simulink model "nmm2d"  (R2025a)
settings: Solver=ode15s  StartTime=0.0  StopTime=20  FixedStep=1e-3  MaxStep=ts_max  RelTol=1e-3  AbsTol=1e-4  EnableMultiTasking=on
values from neighbouring files (symbols this model uses):
  c = 0.05    [nmm2d_mInit.m]
  c_jointstop = 0.3 / (pi/180)    (= 17.1887338539)    [nmm2d_mInit.m]
  D12_F = 0.16    [nmm2d_mInit.m]
  D12_S = L_S    (= 0.5)    [nmm2d_mInit.m]
  D12_T = L_T    (= 0.5)    [nmm2d_mInit.m]
  D1G_F = 0.14    [nmm2d_mInit.m]
  D1G_HAT = 0.35    [nmm2d_mInit.m]
  D1G_S = 0.3    [nmm2d_mInit.m]
  D1G_T = 0.3    [nmm2d_mInit.m]
  DeltaThRef = 5e-3    (= 0.005)    [nmm2d_mInit.m]
  eref = 0.04    [nmm2d_mInit.m]
  FmaxVec = [FmaxSOL FmaxTA FmaxGAS FmaxVAS FmaxHAM FmaxGLU FmaxHFL               FmaxSOL FmaxTA FmaxGAS FmaxVAS FmaxHAM FmaxGLU FmaxHFL]'    [nmm2d_mInit.m]
  g = 9.81    [nmm2d_mInit.m]
  GainDeltaTheta = 2 /100*180/pi    (= 1.14591559026)    [nmm2d_cInit.m]
  GainGAS = 1.1/FmaxGAS    [nmm2d_cInit.m]
  GainGLU = 0.5/FmaxGLU    [nmm2d_cInit.m]
  GainHAM = 0.65/FmaxHAM    [nmm2d_cInit.m]
  GainHAMHFL = 4    [nmm2d_cInit.m]
  GainHFL = 0.5    [nmm2d_cInit.m]
  GainKneOverExt = 2    [nmm2d_cInit.m]
  GainSOL = 1.2/FmaxSOL    [nmm2d_cInit.m]
  GainSOLTA = 0.4/FmaxSOL    [nmm2d_cInit.m]
  GainTA = 1.1    [nmm2d_cInit.m]
  GainVAS = 1.2/FmaxVAS    [nmm2d_cInit.m]
  HAT_CG0 = [-D12_F; 0] + Rot120*[L_S;0] + Rot120*Rot230*[-L_T;0]            + Rot120*Rot230*Rot340*[D1G_HAT;0]    [nmm2d_cInit.m]
  In_F = 0.005    [nmm2d_mInit.m]
  In_HAT = 3    [nmm2d_mInit.m]
  In_S = 0.05    [nmm2d_mInit.m]
  In_T = 0.15    [nmm2d_mInit.m]
  K = 5    [nmm2d_mInit.m]
  k_gx = (2*(m_F+m_S+m_T)+m_HAT)*g/0.1    (= 7848)    [nmm2d_mInit.m]
  k_gy = (2*(m_F+m_S+m_T)+m_HAT)*g/0.01    (= 78480)    [nmm2d_mInit.m]
  k_pressure = m_HAT * 9.81 / DeltaThRef    (= 104967)    [nmm2d_mInit.m]
  K_swing = 0.25    [nmm2d_cInit.m]
  KneePh23Offset = 170*pi/180    (= 2.96705972839)    [nmm2d_cInit.m]
  L_F = 0.2    [nmm2d_mInit.m]
  L_HAT = 0.8    [nmm2d_mInit.m]
  L_S = 0.5    [nmm2d_mInit.m]
  L_T = 0.5    [nmm2d_mInit.m]
  LceOffsetHAM = 0.85    [nmm2d_cInit.m]
  LceOffsetHFL = 0.65    [nmm2d_cInit.m]
  LceOffsetTA = 1-0.5*w    [nmm2d_cInit.m]
  LongDelay = 0.020    (= 0.02)    [nmm2d_cInit.m]
  loptGAS = 0.05    [nmm2d_mInit.m]
  loptGLU = 0.11    [nmm2d_mInit.m]
  loptHAM = 0.10    (= 0.1)    [nmm2d_mInit.m]
  loptHFL = 0.11    [nmm2d_mInit.m]
  loptSOL = 0.04    [nmm2d_mInit.m]
  loptTA = 0.06    [nmm2d_mInit.m]
  loptVAS = 0.08    [nmm2d_mInit.m]
  loptVec = [loptSOL loptTA loptGAS loptVAS loptHAM loptGLU loptHFL               loptSOL loptTA loptGAS loptVAS loptHAM loptGLU loptHFL]'    [nmm2d_mInit.m]
  Lphi120 = 85*pi/180    (= 1.4835298642)    [nmm2d_cInit.m]
  Lphi230 = 175*pi/180    (= 3.05432619099)    [nmm2d_cInit.m]
  Lphi340 = 175*pi/180    (= 3.05432619099)    [nmm2d_cInit.m]
  lslackGAS = 0.40    (= 0.4)    [nmm2d_mInit.m]
  lslackGLU = 0.13    [nmm2d_mInit.m]
  lslackHAM = 0.31    [nmm2d_mInit.m]
  lslackHFL = 0.10    (= 0.1)    [nmm2d_mInit.m]
  lslackSOL = 0.26    [nmm2d_mInit.m]
  lslackTA = 0.24    [nmm2d_mInit.m]
  lslackVAS = 0.23    [nmm2d_mInit.m]
  lslackVec = [lslackSOL lslackTA lslackGAS lslackVAS lslackHAM lslackGLU lslackHFL                 lslackSOL lslackTA lslackGAS lslackVAS lslackHAM lslackGLU lslackHFL]'    [nmm2d_mInit.m]
  m_F = 1.25    [nmm2d_mInit.m]
  m_HAT = 53.5    [nmm2d_mInit.m]
  m_S = 3.5    [nmm2d_mInit.m]
  m_T = 8.5    [nmm2d_mInit.m]
  MidDelay = 0.010    (= 0.01)    [nmm2d_cInit.m]
  mu_slide = 0.8    [nmm2d_mInit.m]
  mu_stick = 0.9    [nmm2d_mInit.m]
  N = 1.5    [nmm2d_mInit.m]
  phi12_LowLimit = 70*pi/180    (= 1.2217304764)    [nmm2d_mInit.m]
  phi12_UpLimit = 130*pi/180    (= 2.26892802759)    [nmm2d_mInit.m]
  phi23_UpLimit = 175*pi/180    (= 3.05432619099)    [nmm2d_mInit.m]
  phi34_UpLimit = 230*pi/180    (= 4.01425727959)    [nmm2d_mInit.m]
  phimaxGASa = 110*pi/180    (= 1.91986217719)    [nmm2d_mInit.m]
  phimaxGASk = 140*pi/180    (= 2.44346095279)    [nmm2d_mInit.m]
  phimaxHAMk = 180*pi/180    (= 3.14159265359)    [nmm2d_mInit.m]
  phimaxSOL = 110*pi/180    (= 1.91986217719)    [nmm2d_mInit.m]
  phimaxTA = 80*pi/180    (= 1.3962634016)    [nmm2d_mInit.m]
  phimaxVAS = 165*pi/180    (= 2.87979326579)    [nmm2d_mInit.m]
  phirefGASa = 80*pi/180    (= 1.3962634016)    [nmm2d_mInit.m]
  phirefGASk = 165*pi/180    (= 2.87979326579)    [nmm2d_mInit.m]
  phirefGLU = 150*pi/180    (= 2.61799387799)    [nmm2d_mInit.m]
  phirefHAMh = 155*pi/180    (= 2.70526034059)    [nmm2d_mInit.m]
  phirefHAMk = 180*pi/180    (= 3.14159265359)    [nmm2d_mInit.m]
  phirefHFL = 180*pi/180    (= 3.14159265359)    [nmm2d_mInit.m]
  phirefSOL = 80*pi/180    (= 1.3962634016)    [nmm2d_mInit.m]
  phirefTA = 110*pi/180    (= 1.91986217719)    [nmm2d_mInit.m]
  phirefVAS = 125*pi/180    (= 2.18166156499)    [nmm2d_mInit.m]
  PosGainGG = 1/(30*pi/180)    (= 1.9098593171)    [nmm2d_cInit.m]
  preA = 0.01    [nmm2d_mInit.m]
  PreStimGAS = 0.01    [nmm2d_cInit.m]
  PreStimGG = 0.05    [nmm2d_cInit.m]
  PreStimGLU = 0.01    [nmm2d_cInit.m]
  PreStimHAM = 0.01    [nmm2d_cInit.m]
  PreStimHFL = 0.01    [nmm2d_cInit.m]
  PreStimSOL = 0.01    [nmm2d_cInit.m]
  PreStimTA = 0.01    [nmm2d_cInit.m]
  PreStimVAS = 0.08    [nmm2d_cInit.m]
  rGASa = 0.05    [nmm2d_mInit.m]
  rGASk = 0.05    [nmm2d_mInit.m]
  rGLU = 0.10    (= 0.1)    [nmm2d_mInit.m]
  rHAMh = 0.08    [nmm2d_mInit.m]
  rHAMk = 0.05    [nmm2d_mInit.m]
  rHFL = 0.10    (= 0.1)    [nmm2d_mInit.m]
  rhoGASa = 0.7    [nmm2d_mInit.m]
  rhoGASk = 0.7    [nmm2d_mInit.m]
  rhoGLU = 0.5    [nmm2d_mInit.m]
  rhoHAMh = 0.7    [nmm2d_mInit.m]
  rhoHAMk = 0.7    [nmm2d_mInit.m]
  rhoHFL = 0.5    [nmm2d_mInit.m]
  rhoSOL = 0.5    [nmm2d_mInit.m]
  rhoTA = 0.7    [nmm2d_mInit.m]
  rhoVAS = 0.7    [nmm2d_mInit.m]
  Rphi120 = 90*pi/180    (= 1.57079632679)    [nmm2d_cInit.m]
  Rphi230 = 175*pi/180    (= 3.05432619099)    [nmm2d_cInit.m]
  Rphi340 = 140*pi/180    (= 2.44346095279)    [nmm2d_cInit.m]
  rSOL = 0.05    [nmm2d_mInit.m]
  rTA = 0.04    [nmm2d_mInit.m]
  rVAS = 0.06    [nmm2d_mInit.m]
  ... (+12 more)
undefined symbols (not defined in the file or in its folder): sgn, X, Y, Z
libraries: sm_lib x70, nesl_utility x67, simulink x27, simulink_extras x6
(part 3 of 5)

== system nmm2d/Body Mechanics Layer/Left Thigh Low ==
  Rotate CG to align body w/ x-y plane : sm_lib/Frames and Transforms/Rigid Transform  RotationMethod=StandardAxis  FollAlignAxisA=+X  BaseAlignAxisA=+Y  FollAlignAxisB=+Y  BaseAlignAxisB=+Z  RotationStandardAxis=+X  RotationAngle=-90  RotationAngleUnits=deg  RotationArbitraryAxis=[0 0 1]  RotationSequenceAxes=FollowerAxes  RotationSequence=XYX  RotationSequenceAngles=[0 0 0]  RotationSequenceAnglesUnits=deg  RotationMatrix=[1 0 0; 0 1 0; 0 0 1]  Quaternion=[1 0 0 0]  TranslationMethod=None  TranslationCartesianOffset=[0.25 0 0]  TranslationCartesianOffsetUnits=m  TranslationStandardAxis=+Y  TranslationStandardOffset=-D1G_HAT  TranslationStandardOffsetUnits=m  TranslationROffset=0  TranslationROffsetUnits=m  TranslationThetaOffset=0  TranslationThetaOffsetUnits=deg  TranslationZOffset=0  TranslationZOffsetUnits=m
  Solid : sm_lib/Body Elements/Cylindrical Solid  CylinderRadius=0.03  CylinderRadiusUnits=m  CylinderLength=L_T*ThPos  CylinderLengthUnits=m  ExportEntireGeometry=off  InertiaType=Custom  BasedOnType=Density  Density=2.7  DensityUnits=g/cm^3  Mass=m_T*ThPos  MassUnits=kg  CenterOfMass=[0 0 (D1G_T-L_T/2)*ThPos]  CenterOfMassUnits=m  MomentsOfInertia=In_T*ThPos^3*[1 1 0]  MomentsOfInertiaUnits=kg*m^2  ProductsOfInertia=[0 0 0]  ProductsOfInertiaUnits=kg*m^2  GraphicType=FromGeometry  MarkerShape=Sphere  MarkerSize=10  GraphicVisPropType=SimpleVisualProperties  GraphicDiffuseColor=[1 0.5 0.5]  GraphicOpacity=1.0  GraphicSpecularColor=[0.5 0.5 0.5 1.0]  GraphicAmbientColor=[0.15 0.15 0.15 1.0]  GraphicEmissiveColor=[0 0 0 1.0]  GraphicShininess=75  DoExposeReferenceFrame=off  SerializedFrames=<Frames><Frame><Id>Frame1</Id><Value><Name>CG</Name><Origin><Source>CenterOfMassFrame</Source><FeatureName></FeatureName></Origin><PrimaryAxis><DefinedDirection>+Z</DefinedDirection><Source>ReferenceFrame</Source><SourceDirection>+Z</SourceDirection><FeatureName></FeatureName></PrimaryAxis><SecondaryAxis><DefinedDirection>+X</DefinedDirection><Source>ReferenceFrame</Source><SourceDirection>+X</SourceDirection><FeatureName></FeatureName></SecondaryAxis></Value></Frame></Frames>
  Transform CG to CS2 : sm_lib/Frames and Transforms/Rigid Transform  RotationMethod=None  FollAlignAxisA=+X  BaseAlignAxisA=+Y  FollAlignAxisB=+Y  BaseAlignAxisB=+Z  RotationStandardAxis=+X  RotationAngle=90  RotationAngleUnits=deg  RotationArbitraryAxis=[0 0 1]  RotationSequenceAxes=FollowerAxes  RotationSequence=XYX  RotationSequenceAngles=[0 0 0]  RotationSequenceAnglesUnits=deg  RotationMatrix=[1 0 0; 0 1 0; 0 0 1]  Quaternion=[1 0 0 0]  TranslationMethod=Cartesian  TranslationCartesianOffset=[ 0 D1G_T*ThPos 0]  TranslationCartesianOffsetUnits=m  TranslationStandardAxis=+Y  TranslationStandardOffset=D1G_T*(1-ThPos)  TranslationStandardOffsetUnits=m  TranslationROffset=0  TranslationROffsetUnits=m  TranslationThetaOffset=0  TranslationThetaOffsetUnits=deg  TranslationZOffset=0  TranslationZOffsetUnits=m
  Transform CS1 to CG : sm_lib/Frames and Transforms/Rigid Transform  RotationMethod=None  FollAlignAxisA=+X  BaseAlignAxisA=+Y  FollAlignAxisB=+Y  BaseAlignAxisB=+Z  RotationStandardAxis=+X  RotationAngle=-90  RotationAngleUnits=deg  RotationArbitraryAxis=[0 0 1]  RotationSequenceAxes=FollowerAxes  RotationSequence=XYX  RotationSequenceAngles=[0 0 0]  RotationSequenceAnglesUnits=deg  RotationMatrix=[1 0 0; 0 1 0; 0 0 1]  Quaternion=[1 0 0 0]  TranslationMethod=Cartesian  TranslationCartesianOffset=[0 (D12_T-D1G_T)*ThPos 0]  TranslationCartesianOffsetUnits=m  TranslationStandardAxis=+Y  TranslationStandardOffset=(D12_T-D1G_T)*(1-ThPos)  TranslationStandardOffsetUnits=m  TranslationROffset=0  TranslationROffsetUnits=m  TranslationThetaOffset=0  TranslationThetaOffsetUnits=deg  TranslationZOffset=0  TranslationZOffsetUnits=m
  CS1 : PMIOPort  Side=Left
  CS2 : PMIOPort  Port=2  Side=Right
  connections:
  Solid/LConn1 -- Rotate CG to align body w/ x-y plane/LConn1
  Transform CG to CS2/LConn1 -- Transform CS1 to CG/RConn1 -- Rotate CG to align body w/ x-y plane/RConn1
  Transform CS1 to CG/LConn1 -- CS1/RConn1
  Transform CG to CS2/RConn1 -- CS2/RConn1

== system nmm2d/Body Mechanics Layer/Right Ball Contact ==
  note: Planar Ground Interaction Model
  vBelt : Inport
  " Body Actuator" : nesl_utility/Simulink-PS Converter  PhysicalDomain=network_engine_domain  SubClassName=ps_input  LeftPortType=input  RightPortType=output  PseudoPeriodic=off  Frequencies=[]  NoiseDistribution=none  NoiseParameters=[]  Unit=N  AffineConversion=off  FilteringAndDerivatives=zero  SimscapeFilterOrder=1  InputFilterTimeConstant=.001  UdotUserProvided=0
  " Body Actuator1" : nesl_utility/Simulink-PS Converter  PhysicalDomain=network_engine_domain  SubClassName=ps_input  LeftPortType=input  RightPortType=output  PseudoPeriodic=off  Frequencies=[]  NoiseDistribution=none  NoiseParameters=[]  Unit=N  AffineConversion=off  FilteringAndDerivatives=zero  SimscapeFilterOrder=1  InputFilterTimeConstant=.001  UdotUserProvided=0
  External Force and Torque : sm_lib/Forces and Torques/External Force and Torque  EnableForceX=on  EnableForceY=on  EnableForceZ=off  EnableForce=off  ForceResolutionFrame=World  EnableTorqueX=off  EnableTorqueY=off  EnableTorqueZ=off  EnableTorque=off  TorqueResolutionFrame=AttachedFrame
  Frame Sensor : sm_lib/Frames and Transforms/Transform Sensor  MeasurementFrame=World  RotationSequence=XYX  SenseAngle=off  SenseAxis=off  SenseQ=off  SenseR=off  SenseRotationSequence=off  SenseOmegaX=off  SenseOmegaY=off  SenseOmegaZ=off  SenseOmega=off  SenseQDot=off  SenseRDot=off  SenseRotationSequenceDot=off  SenseAlphaX=off  SenseAlphaY=off  SenseAlphaZ=off  SenseAlpha=off  SenseQDDot=off  SenseRDDot=off  SenseX=on  SenseY=on  SenseZ=off  SenseXYZ=off  SenseRad=off  SenseAzim=off  SenseDist=off  SenseInc=off  SenseXDot=on  SenseYDot=on  SenseZDot=off  SenseXYZDot=off  SenseRadDot=off  SenseAzimDot=off  SenseDistDot=off  SenseIncDot=off  SenseXDDot=off  SenseYDDot=off  SenseZDDot=off  SenseXYZDDot=off  SenseRadDDot=off  SenseAzimDDot=off  SenseDistDDot=off  SenseIncDDot=off
  Ground Friction Model : Subsystem
  Mux : Mux  Inputs=2
  PS-Simulink Converter : nesl_utility/PS-Simulink Converter  PhysicalDomain=network_engine_domain  SubClassName=ps_output  LeftPortType=input  RightPortType=output  PseudoPeriodic=off  Frequencies=[]  VectorFormat=1-D array  Unit=m  AffineConversion=off
  PS-Simulink Converter1 : nesl_utility/PS-Simulink Converter  PhysicalDomain=network_engine_domain  SubClassName=ps_output  LeftPortType=input  RightPortType=output  PseudoPeriodic=off  Frequencies=[]  VectorFormat=1-D array  Unit=m  AffineConversion=off
  PS-Simulink Converter2 : nesl_utility/PS-Simulink Converter  PhysicalDomain=network_engine_domain  SubClassName=ps_output  LeftPortType=input  RightPortType=output  PseudoPeriodic=off  Frequencies=[]  VectorFormat=1-D array  Unit=m/s  AffineConversion=off
  PS-Simulink Converter3 : nesl_utility/PS-Simulink Converter  PhysicalDomain=network_engine_domain  SubClassName=ps_output  LeftPortType=input  RightPortType=output  PseudoPeriodic=off  Frequencies=[]  VectorFormat=1-D array  Unit=m/s  AffineConversion=off
  Sum : Sum  Inputs=-+|
  Terminator : Terminator
  World Frame : sm_lib/Frames and Transforms/World Frame
  skin contact sensor : simulink/Logic and Bit Operations/Compare To Zero  relop=<=  OutDataTypeStr=boolean
  yGround : Constant  Value=0
  F : PMIOPort  Side=Left
  LHeelCnt : Outport
  GRF [N N] : Outport  Port=2
  wires:
  PS-Simulink Converter2/1 -> Ground Friction Model/4(vx [m/s])
  PS-Simulink Converter/1 -> Ground Friction Model/3(x [m])
  PS-Simulink Converter3/1 -> Ground Friction Model/2(vy [m/s])
  PS-Simulink Converter1/1 -> Sum/2
  Sum/1 -> skin contact sensor/1, Ground Friction Model/1(dy [m])
  yGround/1 -> Sum/1
  Mux/1 -> GRF [N N]/1
  skin contact sensor/1 -> LHeelCnt/1, Ground Friction Model/Enable
  Ground Friction Model/1(Fy_Ground[N]) -> Mux/2, " Body Actuator1"/1
  Ground Friction Model/2(Fx_Friction [N]) -> Mux/1, " Body Actuator"/1
  Ground Friction Model/3(Stiction!) -> Terminator/1
  vBelt/1 -> Ground Friction Model/5(vBelt [m/s])
  connections:
  World Frame/RConn1 -- Frame Sensor/LConn1
  PS-Simulink Converter2/LConn1 -- Frame Sensor/RConn4
  PS-Simulink Converter1/LConn1 -- Frame Sensor/RConn3
  Frame Sensor/RConn2 -- PS-Simulink Converter/LConn1
  PS-Simulink Converter3/LConn1 -- Frame Sensor/RConn5
  External Force and Torque/RConn1 -- Frame Sensor/RConn1 -- F/RConn1
  External Force and Torque/LConn2 -- " Body Actuator1"/RConn1
  External Force and Torque/LConn1 -- " Body Actuator"/RConn1

== system nmm2d/Body Mechanics Layer/Right Heel Contact ==
  note: Planar Ground Interaction Model
  vBelt : Inport
  " Body Actuator" : nesl_utility/Simulink-PS Converter  PhysicalDomain=network_engine_domain  SubClassName=ps_input  LeftPortType=input  RightPortType=output  PseudoPeriodic=off  Frequencies=[]  NoiseDistribution=none  NoiseParameters=[]  Unit=N  AffineConversion=off  FilteringAndDerivatives=zero  SimscapeFilterOrder=1  InputFilterTimeConstant=.001  UdotUserProvided=0
  " Body Actuator1" : nesl_utility/Simulink-PS Converter  PhysicalDomain=network_engine_domain  SubClassName=ps_input  LeftPortType=input  RightPortType=output  PseudoPeriodic=off  Frequencies=[]  NoiseDistribution=none  NoiseParameters=[]  Unit=N  AffineConversion=off  FilteringAndDerivatives=zero  SimscapeFilterOrder=1  InputFilterTimeConstant=.001  UdotUserProvided=0
  External Force and Torque : sm_lib/Forces and Torques/External Force and Torque  EnableForceX=on  EnableForceY=on  EnableForceZ=off  EnableForce=off  ForceResolutionFrame=World  EnableTorqueX=off  EnableTorqueY=off  EnableTorqueZ=off  EnableTorque=off  TorqueResolutionFrame=AttachedFrame
  Frame Sensor : sm_lib/Frames and Transforms/Transform Sensor  MeasurementFrame=World  RotationSequence=XYX  SenseAngle=off  SenseAxis=off  SenseQ=off  SenseR=off  SenseRotationSequence=off  SenseOmegaX=off  SenseOmegaY=off  SenseOmegaZ=off  SenseOmega=off  SenseQDot=off  SenseRDot=off  SenseRotationSequenceDot=off  SenseAlphaX=off  SenseAlphaY=off  SenseAlphaZ=off  SenseAlpha=off  SenseQDDot=off  SenseRDDot=off  SenseX=on  SenseY=on  SenseZ=off  SenseXYZ=off  SenseRad=off  SenseAzim=off  SenseDist=off  SenseInc=off  SenseXDot=on  SenseYDot=on  SenseZDot=off  SenseXYZDot=off  SenseRadDot=off  SenseAzimDot=off  SenseDistDot=off  SenseIncDot=off  SenseXDDot=off  SenseYDDot=off  SenseZDDot=off  SenseXYZDDot=off  SenseRadDDot=off  SenseAzimDDot=off  SenseDistDDot=off  SenseIncDDot=off
  Ground Friction Model : Subsystem
  Mux : Mux  Inputs=2
  PS-Simulink Converter : nesl_utility/PS-Simulink Converter  PhysicalDomain=network_engine_domain  SubClassName=ps_output  LeftPortType=input  RightPortType=output  PseudoPeriodic=off  Frequencies=[]  VectorFormat=1-D array  Unit=m  AffineConversion=off
  PS-Simulink Converter1 : nesl_utility/PS-Simulink Converter  PhysicalDomain=network_engine_domain  SubClassName=ps_output  LeftPortType=input  RightPortType=output  PseudoPeriodic=off  Frequencies=[]  VectorFormat=1-D array  Unit=m  AffineConversion=off
  PS-Simulink Converter2 : nesl_utility/PS-Simulink Converter  PhysicalDomain=network_engine_domain  SubClassName=ps_output  LeftPortType=input  RightPortType=output  PseudoPeriodic=off  Frequencies=[]  VectorFormat=1-D array  Unit=m/s  AffineConversion=off
  PS-Simulink Converter3 : nesl_utility/PS-Simulink Converter  PhysicalDomain=network_engine_domain  SubClassName=ps_output  LeftPortType=input  RightPortType=output  PseudoPeriodic=off  Frequencies=[]  VectorFormat=1-D array  Unit=m/s  AffineConversion=off
  Sum : Sum  Inputs=-+|
  Terminator : Terminator
  World Frame : sm_lib/Frames and Transforms/World Frame
  skin contact sensor : simulink/Logic and Bit Operations/Compare To Zero  relop=<=  OutDataTypeStr=boolean
  yGround : Constant  Value=0
  F : PMIOPort  Side=Left
  LHeelCnt : Outport
  GRF [N N] : Outport  Port=2
  wires:
  vBelt/1 -> Ground Friction Model/5(vBelt [m/s])
  Ground Friction Model/3(Stiction!) -> Terminator/1
  Ground Friction Model/2(Fx_Friction [N]) -> " Body Actuator"/1, Mux/1
  Ground Friction Model/1(Fy_Ground[N]) -> " Body Actuator1"/1, Mux/2
  skin contact sensor/1 -> Ground Friction Model/Enable, LHeelCnt/1
  Mux/1 -> GRF [N N]/1
  yGround/1 -> Sum/1
  Sum/1 -> Ground Friction Model/1(dy [m]), skin contact sensor/1
  PS-Simulink Converter1/1 -> Sum/2
  PS-Simulink Converter3/1 -> Ground Friction Model/2(vy [m/s])
  PS-Simulink Converter/1 -> Ground Friction Model/3(x [m])
  PS-Simulink Converter2/1 -> Ground Friction Model/4(vx [m/s])
  connections:
  External Force and Torque/LConn1 -- " Body Actuator"/RConn1
  External Force and Torque/LConn2 -- " Body Actuator1"/RConn1
  F/RConn1 -- Frame Sensor/RConn1 -- External Force and Torque/RConn1
  PS-Simulink Converter3/LConn1 -- Frame Sensor/RConn5
  Frame Sensor/RConn2 -- PS-Simulink Converter/LConn1
  PS-Simulink Converter1/LConn1 -- Frame Sensor/RConn3
  PS-Simulink Converter2/LConn1 -- Frame Sensor/RConn4
  World Frame/RConn1 -- Frame Sensor/LConn1

== system nmm2d/Body Mechanics Layer/Right Foot ==
  Rotate CG to align body w/ x-y plane : sm_lib/Frames and Transforms/Rigid Transform  RotationMethod=StandardAxis  FollAlignAxisA=+X  BaseAlignAxisA=+Y  FollAlignAxisB=+Y  BaseAlignAxisB=+Z  RotationStandardAxis=+X  RotationAngle=-90  RotationAngleUnits=deg  RotationArbitraryAxis=[0 0 1]  RotationSequenceAxes=FollowerAxes  RotationSequence=XYX  RotationSequenceAngles=[0 0 0]  RotationSequenceAnglesUnits=deg  RotationMatrix=[1 0 0; 0 1 0; 0 0 1]  Quaternion=[1 0 0 0]  TranslationMethod=None  TranslationCartesianOffset=[0.25 0 0]  TranslationCartesianOffsetUnits=m  TranslationStandardAxis=+Y  TranslationStandardOffset=-D1G_HAT  TranslationStandardOffsetUnits=m  TranslationROffset=0  TranslationROffsetUnits=m  TranslationThetaOffset=0  TranslationThetaOffsetUnits=deg  TranslationZOffset=0  TranslationZOffsetUnits=m
  Solid : sm_lib/Body Elements/Cylindrical Solid  CylinderRadius=0.01  CylinderRadiusUnits=m  CylinderLength=L_F  CylinderLengthUnits=m  ExportEntireGeometry=off  InertiaType=Custom  BasedOnType=Density  Density=2.7  DensityUnits=g/cm^3  Mass=m_F  MassUnits=kg  CenterOfMass=[0 0 D1G_F-L_F/2]  CenterOfMassUnits=m  MomentsOfInertia=In_F*[1 1 0]  MomentsOfInertiaUnits=kg*m^2  ProductsOfInertia=[0 0 0]  ProductsOfInertiaUnits=kg*m^2  GraphicType=FromGeometry  MarkerShape=Sphere  MarkerSize=10  GraphicVisPropType=SimpleVisualProperties  GraphicDiffuseColor=[1 0.5 0.5]  GraphicOpacity=1.0  GraphicSpecularColor=[0.5 0.5 0.5 1.0]  GraphicAmbientColor=[0.15 0.15 0.15 1.0]  GraphicEmissiveColor=[0 0 0 1.0]  GraphicShininess=75  DoExposeReferenceFrame=off  SerializedFrames=<Frames><Frame><Id>Frame1</Id><Value><Name>CG</Name><Origin><Source>CenterOfMassFrame</Source><FeatureName></FeatureName></Origin><PrimaryAxis><DefinedDirection>+Z</DefinedDirection><Source>ReferenceFrame</Source><SourceDirection>+Z</SourceDirection><FeatureName></FeatureName></PrimaryAxis><SecondaryAxis><DefinedDirection>+X</DefinedDirection><Source>ReferenceFrame</Source><SourceDirection>+X</SourceDirection><FeatureName></FeatureName></SecondaryAxis></Value></Frame></Frames>
  Transform CG to CS2 : sm_lib/Frames and Transforms/Rigid Transform  RotationMethod=None  FollAlignAxisA=+X  BaseAlignAxisA=+Y  FollAlignAxisB=+Y  BaseAlignAxisB=+Z  RotationStandardAxis=+X  RotationAngle=90  RotationAngleUnits=deg  RotationArbitraryAxis=[0 0 1]  RotationSequenceAxes=FollowerAxes  RotationSequence=XYX  RotationSequenceAngles=[0 0 0]  RotationSequenceAnglesUnits=deg  RotationMatrix=[1 0 0; 0 1 0; 0 0 1]  Quaternion=[1 0 0 0]  TranslationMethod=Cartesian  TranslationCartesianOffset=[ 0 D1G_F 0]  TranslationCartesianOffsetUnits=m  TranslationStandardAxis=+Y  TranslationStandardOffset=D1G_T*(1-ThPos)  TranslationStandardOffsetUnits=m  TranslationROffset=0  TranslationROffsetUnits=m  TranslationThetaOffset=0  TranslationThetaOffsetUnits=deg  TranslationZOffset=0  TranslationZOffsetUnits=m
  Transform CS1 to CG : sm_lib/Frames and Transforms/Rigid Transform  RotationMethod=None  FollAlignAxisA=+X  BaseAlignAxisA=+Y  FollAlignAxisB=+Y  BaseAlignAxisB=+Z  RotationStandardAxis=+X  RotationAngle=-90  RotationAngleUnits=deg  RotationArbitraryAxis=[0 0 1]  RotationSequenceAxes=FollowerAxes  RotationSequence=XYX  RotationSequenceAngles=[0 0 0]  RotationSequenceAnglesUnits=deg  RotationMatrix=[1 0 0; 0 1 0; 0 0 1]  Quaternion=[1 0 0 0]  TranslationMethod=Cartesian  TranslationCartesianOffset=[0 (D12_F-D1G_F) 0]  TranslationCartesianOffsetUnits=m  TranslationStandardAxis=+Y  TranslationStandardOffset=(D12_T-D1G_T)*(1-ThPos)  TranslationStandardOffsetUnits=m  TranslationROffset=0  TranslationROffsetUnits=m  TranslationThetaOffset=0  TranslationThetaOffsetUnits=deg  TranslationZOffset=0  TranslationZOffsetUnits=m
  Transform CS1 to CS3 : sm_lib/Frames and Transforms/Rigid Transform  RotationMethod=None  FollAlignAxisA=+X  BaseAlignAxisA=+Y  FollAlignAxisB=+Y  BaseAlignAxisB=+Z  RotationStandardAxis=+X  RotationAngle=-90  RotationAngleUnits=deg  RotationArbitraryAxis=[0 0 1]  RotationSequenceAxes=FollowerAxes  RotationSequence=XYX  RotationSequenceAngles=[0 0 0]  RotationSequenceAnglesUnits=deg  RotationMatrix=[1 0 0; 0 1 0; 0 0 1]  Quaternion=[1 0 0 0]  TranslationMethod=Cartesian  TranslationCartesianOffset=[0 -(L_F-D12_F) 0]  TranslationCartesianOffsetUnits=m  TranslationStandardAxis=+Y  TranslationStandardOffset=(D12_T-D1G_T)*(1-ThPos)  TranslationStandardOffsetUnits=m  TranslationROffset=0  TranslationROffsetUnits=m  TranslationThetaOffset=0  TranslationThetaOffsetUnits=deg  TranslationZOffset=0  TranslationZOffsetUnits=m
  CS1 : PMIOPort  Side=Left
  CS2 : PMIOPort  Port=2  Side=Right
  CS3 : PMIOPort  Port=3  Side=Left
  connections:
  Transform CS1 to CS3/RConn1 -- CS3/RConn1
  Solid/LConn1 -- Rotate CG to align body w/ x-y plane/LConn1
  Rotate CG to align body w/ x-y plane/RConn1 -- Transform CG to CS2/LConn1 -- Transform CS1 to CG/RConn1
  CS1/RConn1 -- Transform CS1 to CS3/LConn1 -- Transform CS1 to CG/LConn1
  Transform CG to CS2/RConn1 -- CS2/RConn1

== system nmm2d/Body Mechanics Layer/Right Force Plate ==
  "GRF_Ball [N N] " : Inport
  GRF_Heel [N N] : Inport  Port=2
  Enable : EnablePort  StatesWhenEnabling=reset
  Fcn : Fcn  Expr=u(1)/(u(2)+eps)
  Mux : Mux  Inputs=3
  Mux1 : Mux  Inputs=2
  Selector : Selector  InputPortWidth=2  IndexOptions=Index vector (dialog)  Indices=2  OutputSizes=1
  Selector1 : Selector  InputPortWidth=2  IndexOptions=Index vector (dialog)  Indices=2  OutputSizes=1
  Sum1 : Sum
  GRFs : Outport  OutputWhenDisabled=reset  InitialOutput=0
  COP : Outport  Port=2  OutputWhenDisabled=reset  InitialOutput=0
  wires:
  Fcn/1 -> COP/1
  Mux1/1 -> Fcn/1
  Mux/1 -> GRFs/1
  Sum1/1 -> Selector/1, Mux/2
  GRF_Heel [N N]/1 -> Mux/3, Sum1/2
  "GRF_Ball [N N] "/1 -> Selector1/1, Mux/1, Sum1/1
  Selector1/1 -> Mux1/1
  Selector/1 -> Mux1/2

== system nmm2d/Body Mechanics Layer/Right Shank ==
  Rotate CG to align body w/ x-y plane : sm_lib/Frames and Transforms/Rigid Transform  RotationMethod=StandardAxis  FollAlignAxisA=+X  BaseAlignAxisA=+Y  FollAlignAxisB=+Y  BaseAlignAxisB=+Z  RotationStandardAxis=+X  RotationAngle=-90  RotationAngleUnits=deg  RotationArbitraryAxis=[0 0 1]  RotationSequenceAxes=FollowerAxes  RotationSequence=XYX  RotationSequenceAngles=[0 0 0]  RotationSequenceAnglesUnits=deg  RotationMatrix=[1 0 0; 0 1 0; 0 0 1]  Quaternion=[1 0 0 0]  TranslationMethod=None  TranslationCartesianOffset=[0.25 0 0]  TranslationCartesianOffsetUnits=m  TranslationStandardAxis=+Y  TranslationStandardOffset=-D1G_HAT  TranslationStandardOffsetUnits=m  TranslationROffset=0  TranslationROffsetUnits=m  TranslationThetaOffset=0  TranslationThetaOffsetUnits=deg  TranslationZOffset=0  TranslationZOffsetUnits=m
  Solid : sm_lib/Body Elements/Cylindrical Solid  CylinderRadius=0.02  CylinderRadiusUnits=m  CylinderLength=L_S  CylinderLengthUnits=m  ExportEntireGeometry=off  InertiaType=Custom  BasedOnType=Density  Density=2.7  DensityUnits=g/cm^3  Mass=m_S  MassUnits=kg  CenterOfMass=[0 0 L_S/2-D1G_S]  CenterOfMassUnits=m  MomentsOfInertia=In_S*[1 1 0]  MomentsOfInertiaUnits=kg*m^2  ProductsOfInertia=[0 0 0]  ProductsOfInertiaUnits=kg*m^2  GraphicType=FromGeometry  MarkerShape=Sphere  MarkerSize=10  GraphicVisPropType=SimpleVisualProperties  GraphicDiffuseColor=[1 0.5 0.5]  GraphicOpacity=1.0  GraphicSpecularColor=[0.5 0.5 0.5 1.0]  GraphicAmbientColor=[0.15 0.15 0.15 1.0]  GraphicEmissiveColor=[0 0 0 1.0]  GraphicShininess=75  DoExposeReferenceFrame=off  SerializedFrames=<Frames><Frame><Id>Frame1</Id><Value><Name>CG</Name><Origin><Source>CenterOfMassFrame</Source><FeatureName></FeatureName></Origin><PrimaryAxis><DefinedDirection>+Z</DefinedDirection><Source>ReferenceFrame</Source><SourceDirection>+Z</SourceDirection><FeatureName></FeatureName></PrimaryAxis><SecondaryAxis><DefinedDirection>+X</DefinedDirection><Source>ReferenceFrame</Source><SourceDirection>+X</SourceDirection><FeatureName></FeatureName></SecondaryAxis></Value></Frame></Frames>
  Transform CG to CS2 : sm_lib/Frames and Transforms/Rigid Transform  RotationMethod=None  FollAlignAxisA=+X  BaseAlignAxisA=+Y  FollAlignAxisB=+Y  BaseAlignAxisB=+Z  RotationStandardAxis=+X  RotationAngle=90  RotationAngleUnits=deg  RotationArbitraryAxis=[0 0 1]  RotationSequenceAxes=FollowerAxes  RotationSequence=XYX  RotationSequenceAngles=[0 0 0]  RotationSequenceAnglesUnits=deg  RotationMatrix=[1 0 0; 0 1 0; 0 0 1]  Quaternion=[1 0 0 0]  TranslationMethod=Cartesian  TranslationCartesianOffset=[ 0 -D1G_S 0]  TranslationCartesianOffsetUnits=m  TranslationStandardAxis=+Y  TranslationStandardOffset=D1G_T*(1-ThPos)  TranslationStandardOffsetUnits=m  TranslationROffset=0  TranslationROffsetUnits=m  TranslationThetaOffset=0  TranslationThetaOffsetUnits=deg  TranslationZOffset=0  TranslationZOffsetUnits=m
  Transform CS1 to CG : sm_lib/Frames and Transforms/Rigid Transform  RotationMethod=None  FollAlignAxisA=+X  BaseAlignAxisA=+Y  FollAlignAxisB=+Y  BaseAlignAxisB=+Z  RotationStandardAxis=+X  RotationAngle=-90  RotationAngleUnits=deg  RotationArbitraryAxis=[0 0 1]  RotationSequenceAxes=FollowerAxes  RotationSequence=XYX  RotationSequenceAngles=[0 0 0]  RotationSequenceAnglesUnits=deg  RotationMatrix=[1 0 0; 0 1 0; 0 0 1]  Quaternion=[1 0 0 0]  TranslationMethod=Cartesian  TranslationCartesianOffset=[0 -(D12_S-D1G_S) 0]  TranslationCartesianOffsetUnits=m  TranslationStandardAxis=+Y  TranslationStandardOffset=(D12_T-D1G_T)*(1-ThPos)  TranslationStandardOffsetUnits=m  TranslationROffset=0  TranslationROffsetUnits=m  TranslationThetaOffset=0  TranslationThetaOffsetUnits=deg  TranslationZOffset=0  TranslationZOffsetUnits=m
  CS1 : PMIOPort  Side=Left
  CS2 : PMIOPort  Port=2  Side=Right
  connections:
  Transform CG to CS2/RConn1 -- CS2/RConn1
  Transform CS1 to CG/LConn1 -- CS1/RConn1
  Rotate CG to align body w/ x-y plane/RConn1 -- Transform CS1 to CG/RConn1 -- Transform CG to CS2/LConn1
  Solid/LConn1 -- Rotate CG to align body w/ x-y plane/LConn1

== system nmm2d/Body Mechanics Layer/Right Thigh Sensor Sheet ==
  note: Inner Segment Pressure Sheet
  Gain3 : Gain  Gain=k_pressure
  Gain4 : Gain  Gain=1/v_max_pressure
  Inner Thigh Shift Joint : sm_lib/Joints/Prismatic Joint  JointMode=Normal  CompositeWrenchDir=FollowerOnBase  CompositeWrenchFrame=BaseFrame  SenseConstraintForce=off  SenseConstraintTorque=off  SenseTotalForce=off  SenseTotalTorque=off  PositionTargetSpecify=on  PositionTargetPriority=High  PositionTargetValue=0  PositionTargetValueUnits=m  VelocityTargetSpecify=on  VelocityTargetPriority=High  VelocityTargetValue=0  VelocityTargetValueUnits=m/s  EquilibriumPosition=0  EquilibriumPositionUnits=m  SpringStiffness=0  SpringStiffnessUnits=N/m  DampingCoefficient=0  DampingCoefficientUnits=N/(m/s)  LowerLimitSpecify=off  LowerLimitBound=-1  LowerLimitBoundUnits=m  LowerLimitStiffness=1e6  LowerLimitStiffnessUnits=N/m  LowerLimitDamping=1e3  LowerLimitDampingUnits=N/(m/s)  LowerLimitTransitionRegionWidth=1e-4  LowerLimitTransitionRegionWidthUnits=m  UpperLimitSpecify=off  UpperLimitBound=1  UpperLimitBoundUnits=m  UpperLimitStiffness=1e6  UpperLimitStiffnessUnits=N/m  UpperLimitDamping=1e3  UpperLimitDampingUnits=N/(m/s)  UpperLimitTransitionRegionWidth=1e-4  UpperLimitTransitionRegionWidthUnits=m  TorqueActuationMode=InputTorque  MotionActuationMode=ComputedMotion  SensePosition=on  SenseVelocity=on  SenseAcceleration=off  SenseTorqueForce=off  SenseLowerLimitTorqueForce=off  SenseUpperLimitTorqueForce=off
  Mux1 : Mux  Inputs=2
  Pressure Sheet Reaction Force : Fcn  Expr=-u(1) * (1+sgn(u(1))*u(2))
  Rotate back to y-axis : sm_lib/Frames and Transforms/Rigid Transform  RotationMethod=StandardAxis  FollAlignAxisA=+X  BaseAlignAxisA=+Y  FollAlignAxisB=+Y  BaseAlignAxisB=+Z  RotationStandardAxis=+X  RotationAngle=-90  RotationAngleUnits=deg  RotationArbitraryAxis=[0 0 1]  RotationSequenceAxes=FollowerAxes  RotationSequence=XYX  RotationSequenceAngles=[0 0 0]  RotationSequenceAnglesUnits=deg  RotationMatrix=[1 0 0; 0 1 0; 0 0 1]  Quaternion=[1 0 0 0]  TranslationMethod=None  TranslationCartesianOffset=[0 0 0]  TranslationCartesianOffsetUnits=m  TranslationStandardAxis=+Z  TranslationStandardOffset=0  TranslationStandardOffsetUnits=m  TranslationROffset=0  TranslationROffsetUnits=m  TranslationThetaOffset=0  TranslationThetaOffsetUnits=deg  TranslationZOffset=0  TranslationZOffsetUnits=m
  Rotate into z-axis : sm_lib/Frames and Transforms/Rigid Transform  RotationMethod=StandardAxis  FollAlignAxisA=+X  BaseAlignAxisA=+Y  FollAlignAxisB=+Y  BaseAlignAxisB=+Z  RotationStandardAxis=+X  RotationAngle=90  RotationAngleUnits=deg  RotationArbitraryAxis=[0 0 1]  RotationSequenceAxes=FollowerAxes  RotationSequence=XYX  RotationSequenceAngles=[0 0 0]  RotationSequenceAnglesUnits=deg  RotationMatrix=[1 0 0; 0 1 0; 0 0 1]  Quaternion=[1 0 0 0]  TranslationMethod=None  TranslationCartesianOffset=[0 0 0]  TranslationCartesianOffsetUnits=m  TranslationStandardAxis=+Z  TranslationStandardOffset=0  TranslationStandardOffsetUnits=m  TranslationROffset=0  TranslationROffsetUnits=m  TranslationThetaOffset=0  TranslationThetaOffsetUnits=deg  TranslationZOffset=0  TranslationZOffsetUnits=m
  Thigh Actuator : nesl_utility/Simulink-PS Converter  PhysicalDomain=network_engine_domain  SubClassName=ps_input  LeftPortType=input  RightPortType=output  PseudoPeriodic=off  Frequencies=[]  NoiseDistribution=none  NoiseParameters=[]  Unit=N  AffineConversion=off  FilteringAndDerivatives=zero  SimscapeFilterOrder=1  InputFilterTimeConstant=.001  UdotUserProvided=0
  Thigh Pos Sensor : nesl_utility/PS-Simulink Converter  PhysicalDomain=network_engine_domain  SubClassName=ps_output  LeftPortType=input  RightPortType=output  PseudoPeriodic=off  Frequencies=[]  VectorFormat=1-D array  Unit=m  AffineConversion=off
  Thigh Vel Sensor : nesl_utility/PS-Simulink Converter  PhysicalDomain=network_engine_domain  SubClassName=ps_output  LeftPortType=input  RightPortType=output  PseudoPeriodic=off  Frequencies=[]  VectorFormat=1-D array  Unit=m/s  AffineConversion=off
  F : PMIOPort  Side=Right
  B : PMIOPort  Port=2  Side=Left
  dx : Outport
  wires:
  Gain3/1 -> Mux1/1
  Gain4/1 -> Mux1/2
  Mux1/1 -> Pressure Sheet Reaction Force/1
  Thigh Vel Sensor/1 -> Gain4/1
  Pressure Sheet Reaction Force/1 -> Thigh Actuator/1
  Thigh Pos Sensor/1 -> Gain3/1, dx/1
  connections:
  F/RConn1 -- Rotate back to y-axis/RConn1
  B/RConn1 -- Rotate into z-axis/LConn1
  Inner Thigh Shift Joint/RConn2 -- Thigh Pos Sensor/LConn1
  Thigh Vel Sensor/LConn1 -- Inner Thigh Shift Joint/RConn3
  Thigh Actuator/RConn1 -- Inner Thigh Shift Joint/LConn2
  Rotate into z-axis/RConn1 -- Inner Thigh Shift Joint/LConn1
  Rotate back to y-axis/LConn1 -- Inner Thigh Shift Joint/RConn1

== system nmm2d/Body Mechanics Layer/Right Thigh High ==
  Rotate CG to align body w/ x-y plane : sm_lib/Frames and Transforms/Rigid Transform  RotationMethod=StandardAxis  FollAlignAxisA=+X  BaseAlignAxisA=+Y  FollAlignAxisB=+Y  BaseAlignAxisB=+Z  RotationStandardAxis=+X  RotationAngle=-90  RotationAngleUnits=deg  RotationArbitraryAxis=[0 0 1]  RotationSequenceAxes=FollowerAxes  RotationSequence=XYX  RotationSequenceAngles=[0 0 0]  RotationSequenceAnglesUnits=deg  RotationMatrix=[1 0 0; 0 1 0; 0 0 1]  Quaternion=[1 0 0 0]  TranslationMethod=None  TranslationCartesianOffset=[0.25 0 0]  TranslationCartesianOffsetUnits=m  TranslationStandardAxis=+Y  TranslationStandardOffset=-D1G_HAT  TranslationStandardOffsetUnits=m  TranslationROffset=0  TranslationROffsetUnits=m  TranslationThetaOffset=0  TranslationThetaOffsetUnits=deg  TranslationZOffset=0  TranslationZOffsetUnits=m
  Solid : sm_lib/Body Elements/Cylindrical Solid  CylinderRadius=0.03  CylinderRadiusUnits=m  CylinderLength=L_T*(1-ThPos)  CylinderLengthUnits=m  ExportEntireGeometry=off  InertiaType=Custom  BasedOnType=Density  Density=2.7  DensityUnits=g/cm^3  Mass=m_T*(1-ThPos)  MassUnits=kg  CenterOfMass=[0 0 (D1G_T-L_T/2)*(1-ThPos)]  CenterOfMassUnits=m  MomentsOfInertia=In_T*(1-ThPos)^3*[1 1 0]  MomentsOfInertiaUnits=kg*m^2  ProductsOfInertia=[0 0 0]  ProductsOfInertiaUnits=kg*m^2  GraphicType=FromGeometry  MarkerShape=Sphere  MarkerSize=10  GraphicVisPropType=SimpleVisualProperties  GraphicDiffuseColor=[1 0.5 0.5]  GraphicOpacity=1.0  GraphicSpecularColor=[0.5 0.5 0.5 1.0]  GraphicAmbientColor=[0.15 0.15 0.15 1.0]  GraphicEmissiveColor=[0 0 0 1.0]  GraphicShininess=75  DoExposeReferenceFrame=off  SerializedFrames=<Frames><Frame><Id>Frame1</Id><Value><Name>CG</Name><Origin><Source>CenterOfMassFrame</Source><FeatureName></FeatureName></Origin><PrimaryAxis><DefinedDirection>+Z</DefinedDirection><Source>ReferenceFrame</Source><SourceDirection>+Z</SourceDirection><FeatureName></FeatureName></PrimaryAxis><SecondaryAxis><DefinedDirection>+X</DefinedDirection><Source>ReferenceFrame</Source><SourceDirection>+X</SourceDirection><FeatureName></FeatureName></SecondaryAxis></Value></Frame></Frames>
  Transform CG to CS2 : sm_lib/Frames and Transforms/Rigid Transform  RotationMethod=None  FollAlignAxisA=+X  BaseAlignAxisA=+Y  FollAlignAxisB=+Y  BaseAlignAxisB=+Z  RotationStandardAxis=+X  RotationAngle=90  RotationAngleUnits=deg  RotationArbitraryAxis=[0 0 1]  RotationSequenceAxes=FollowerAxes  RotationSequence=XYX  RotationSequenceAngles=[0 0 0]  RotationSequenceAnglesUnits=deg  RotationMatrix=[1 0 0; 0 1 0; 0 0 1]  Quaternion=[1 0 0 0]  TranslationMethod=Cartesian  TranslationCartesianOffset=[ 0 D1G_T*(1-ThPos) 0]  TranslationCartesianOffsetUnits=m  TranslationStandardAxis=+Y  TranslationStandardOffset=D1G_T*(1-ThPos)  TranslationStandardOffsetUnits=m  TranslationROffset=0  TranslationROffsetUnits=m  TranslationThetaOffset=0  TranslationThetaOffsetUnits=deg  TranslationZOffset=0  TranslationZOffsetUnits=m
  Transform CS1 to CG : sm_lib/Frames and Transforms/Rigid Transform  RotationMethod=None  FollAlignAxisA=+X  BaseAlignAxisA=+Y  FollAlignAxisB=+Y  BaseAlignAxisB=+Z  RotationStandardAxis=+X  RotationAngle=-90  RotationAngleUnits=deg  RotationArbitraryAxis=[0 0 1]  RotationSequenceAxes=FollowerAxes  RotationSequence=XYX  RotationSequenceAngles=[0 0 0]  RotationSequenceAnglesUnits=deg  RotationMatrix=[1 0 0; 0 1 0; 0 0 1]  Quaternion=[1 0 0 0]  TranslationMethod=Cartesian  TranslationCartesianOffset=[0 (D12_T-D1G_T)*(1-ThPos) 0]  TranslationCartesianOffsetUnits=m  TranslationStandardAxis=+Y  TranslationStandardOffset=(D12_T-D1G_T)*(1-ThPos)  TranslationStandardOffsetUnits=m  TranslationROffset=0  TranslationROffsetUnits=m  TranslationThetaOffset=0  TranslationThetaOffsetUnits=deg  TranslationZOffset=0  TranslationZOffsetUnits=m
  CS1 : PMIOPort  Side=Left
  CS2 : PMIOPort  Port=2  Side=Right
  connections:
  Solid/LConn1 -- Rotate CG to align body w/ x-y plane/LConn1
  Transform CG to CS2/LConn1 -- Transform CS1 to CG/RConn1 -- Rotate CG to align body w/ x-y plane/RConn1
  Transform CS1 to CG/LConn1 -- CS1/RConn1
  Transform CG to CS2/RConn1 -- CS2/RConn1

== system nmm2d/Body Mechanics Layer/Right Thigh Low ==
  Rotate CG to align body w/ x-y plane : sm_lib/Frames and Transforms/Rigid Transform  RotationMethod=StandardAxis  FollAlignAxisA=+X  BaseAlignAxisA=+Y  FollAlignAxisB=+Y  BaseAlignAxisB=+Z  RotationStandardAxis=+X  RotationAngle=-90  RotationAngleUnits=deg  RotationArbitraryAxis=[0 0 1]  RotationSequenceAxes=FollowerAxes  RotationSequence=XYX  RotationSequenceAngles=[0 0 0]  RotationSequenceAnglesUnits=deg  RotationMatrix=[1 0 0; 0 1 0; 0 0 1]  Quaternion=[1 0 0 0]  TranslationMethod=None  TranslationCartesianOffset=[0.25 0 0]  TranslationCartesianOffsetUnits=m  TranslationStandardAxis=+Y  TranslationStandardOffset=-D1G_HAT  TranslationStandardOffsetUnits=m  TranslationROffset=0  TranslationROffsetUnits=m  TranslationThetaOffset=0  TranslationThetaOffsetUnits=deg  TranslationZOffset=0  TranslationZOffsetUnits=m
  Solid : sm_lib/Body Elements/Cylindrical Solid  CylinderRadius=0.03  CylinderRadiusUnits=m  CylinderLength=L_T*ThPos  CylinderLengthUnits=m  ExportEntireGeometry=off  InertiaType=Custom  BasedOnType=Density  Density=2.7  DensityUnits=g/cm^3  Mass=m_T*ThPos  MassUnits=kg  CenterOfMass=[0 0 (D1G_T-L_T/2)*ThPos]  CenterOfMassUnits=m  MomentsOfInertia=In_T*ThPos^3*[1 1 0]  MomentsOfInertiaUnits=kg*m^2  ProductsOfInertia=[0 0 0]  ProductsOfInertiaUnits=kg*m^2  GraphicType=FromGeometry  MarkerShape=Sphere  MarkerSize=10  GraphicVisPropType=SimpleVisualProperties  GraphicDiffuseColor=[1 0.5 0.5]  GraphicOpacity=1.0  GraphicSpecularColor=[0.5 0.5 0.5 1.0]  GraphicAmbientColor=[0.15 0.15 0.15 1.0]  GraphicEmissiveColor=[0 0 0 1.0]  GraphicShininess=75  DoExposeReferenceFrame=off  SerializedFrames=<Frames><Frame><Id>Frame1</Id><Value><Name>CG</Name><Origin><Source>CenterOfMassFrame</Source><FeatureName></FeatureName></Origin><PrimaryAxis><DefinedDirection>+Z</DefinedDirection><Source>ReferenceFrame</Source><SourceDirection>+Z</SourceDirection><FeatureName></FeatureName></PrimaryAxis><SecondaryAxis><DefinedDirection>+X</DefinedDirection><Source>ReferenceFrame</Source><SourceDirection>+X</SourceDirection><FeatureName></FeatureName></SecondaryAxis></Value></Frame></Frames>
  Transform CG to CS2 : sm_lib/Frames and Transforms/Rigid Transform  RotationMethod=None  FollAlignAxisA=+X  BaseAlignAxisA=+Y  FollAlignAxisB=+Y  BaseAlignAxisB=+Z  RotationStandardAxis=+X  RotationAngle=90  RotationAngleUnits=deg  RotationArbitraryAxis=[0 0 1]  RotationSequenceAxes=FollowerAxes  RotationSequence=XYX  RotationSequenceAngles=[0 0 0]  RotationSequenceAnglesUnits=deg  RotationMatrix=[1 0 0; 0 1 0; 0 0 1]  Quaternion=[1 0 0 0]  TranslationMethod=Cartesian  TranslationCartesianOffset=[ 0 D1G_T*ThPos 0]  TranslationCartesianOffsetUnits=m  TranslationStandardAxis=+Y  TranslationStandardOffset=D1G_T*(1-ThPos)  TranslationStandardOffsetUnits=m  TranslationROffset=0  TranslationROffsetUnits=m  TranslationThetaOffset=0  TranslationThetaOffsetUnits=deg  TranslationZOffset=0  TranslationZOffsetUnits=m
  Transform CS1 to CG : sm_lib/Frames and Transforms/Rigid Transform  RotationMethod=None  FollAlignAxisA=+X  BaseAlignAxisA=+Y  FollAlignAxisB=+Y  BaseAlignAxisB=+Z  RotationStandardAxis=+X  RotationAngle=-90  RotationAngleUnits=deg  RotationArbitraryAxis=[0 0 1]  RotationSequenceAxes=FollowerAxes  RotationSequence=XYX  RotationSequenceAngles=[0 0 0]  RotationSequenceAnglesUnits=deg  RotationMatrix=[1 0 0; 0 1 0; 0 0 1]  Quaternion=[1 0 0 0]  TranslationMethod=Cartesian  TranslationCartesianOffset=[0 (D12_T-D1G_T)*ThPos 0]  TranslationCartesianOffsetUnits=m  TranslationStandardAxis=+Y  TranslationStandardOffset=(D12_T-D1G_T)*(1-ThPos)  TranslationStandardOffsetUnits=m  TranslationROffset=0  TranslationROffsetUnits=m  TranslationThetaOffset=0  TranslationThetaOffsetUnits=deg  TranslationZOffset=0  TranslationZOffsetUnits=m
  CS1 : PMIOPort  Side=Left
  CS2 : PMIOPort  Port=2  Side=Right
  connections:
  Transform CG to CS2/RConn1 -- CS2/RConn1
  Transform CS1 to CG/LConn1 -- CS1/RConn1
  Rotate CG to align body w/ x-y plane/RConn1 -- Transform CS1 to CG/RConn1 -- Transform CG to CS2/LConn1
  Solid/LConn1 -- Rotate CG to align body w/ x-y plane/LConn1

== system nmm2d/Body Mechanics Layer/body sensor ==
  Frame Sensor : sm_lib/Frames and Transforms/Transform Sensor  MeasurementFrame=World  RotationSequence=XYX  SenseAngle=off  SenseAxis=off  SenseQ=off  SenseR=off  SenseRotationSequence=off  SenseOmegaX=off  SenseOmegaY=off  SenseOmegaZ=off  SenseOmega=off  SenseQDot=off  SenseRDot=off  SenseRotationSequenceDot=off  SenseAlphaX=off  SenseAlphaY=off  SenseAlphaZ=off  SenseAlpha=off  SenseQDDot=off  SenseRDDot=off  SenseX=on  SenseY=on  SenseZ=on  SenseXYZ=off  SenseRad=off  SenseAzim=off  SenseDist=off  SenseInc=off  SenseXDot=on  SenseYDot=on  SenseZDot=on  SenseXYZDot=off  SenseRadDot=off  SenseAzimDot=off  SenseDistDot=off  SenseIncDot=off  SenseXDDot=off  SenseYDDot=off  SenseZDDot=off  SenseXYZDDot=off  SenseRadDDot=off  SenseAzimDDot=off  SenseDistDDot=off  SenseIncDDot=off
  Mux : Mux  Inputs=3
  Mux1 : Mux  Inputs=3
  PS-Simulink Converter : nesl_utility/PS-Simulink Converter  PhysicalDomain=network_engine_domain  SubClassName=ps_output  LeftPortType=input  RightPortType=output  PseudoPeriodic=off  Frequencies=[]  VectorFormat=1-D array  Unit=m  AffineConversion=off
  PS-Simulink Converter1 : nesl_utility/PS-Simulink Converter  PhysicalDomain=network_engine_domain  SubClassName=ps_output  LeftPortType=input  RightPortType=output  PseudoPeriodic=off  Frequencies=[]  VectorFormat=1-D array  Unit=m  AffineConversion=off
  PS-Simulink Converter2 : nesl_utility/PS-Simulink Converter  PhysicalDomain=network_engine_domain  SubClassName=ps_output  LeftPortType=input  RightPortType=output  PseudoPeriodic=off  Frequencies=[]  VectorFormat=1-D array  Unit=m/s  AffineConversion=off
  PS-Simulink Converter3 : nesl_utility/PS-Simulink Converter  PhysicalDomain=network_engine_domain  SubClassName=ps_output  LeftPortType=input  RightPortType=output  PseudoPeriodic=off  Frequencies=[]  VectorFormat=1-D array  Unit=m/s  AffineConversion=off
  PS-Simulink Converter4 : nesl_utility/PS-Simulink Converter  PhysicalDomain=network_engine_domain  SubClassName=ps_output  LeftPortType=input  RightPortType=output  PseudoPeriodic=off  Frequencies=[]  VectorFormat=1-D array  Unit=m  AffineConversion=off
  PS-Simulink Converter5 : nesl_utility/PS-Simulink Converter  PhysicalDomain=network_engine_domain  SubClassName=ps_output  LeftPortType=input  RightPortType=output  PseudoPeriodic=off  Frequencies=[]  VectorFormat=1-D array  Unit=m/s  AffineConversion=off
  World Frame : sm_lib/Frames and Transforms/World Frame
  frame : PMIOPort  Side=Left
  p [m x3] : Outport
  v [m/s x3] : Outport  Port=2
  wires:
  PS-Simulink Converter1/1 -> Mux/2
  PS-Simulink Converter/1 -> Mux/1
  PS-Simulink Converter2/1 -> Mux1/1
  PS-Simulink Converter3/1 -> Mux1/2
  Mux1/1 -> v [m/s x3]/1
  Mux/1 -> p [m x3]/1
  PS-Simulink Converter4/1 -> Mux/3
  PS-Simulink Converter5/1 -> Mux1/3
  connections:
  Frame Sensor/RConn1 -- frame/RConn1
  World Frame/RConn1 -- Frame Sensor/LConn1
  Frame Sensor/RConn2 -- PS-Simulink Converter/LConn1
  PS-Simulink Converter1/LConn1 -- Frame Sensor/RConn3
  PS-Simulink Converter2/LConn1 -- Frame Sensor/RConn5
  PS-Simulink Converter3/LConn1 -- Frame Sensor/RConn6
  PS-Simulink Converter4/LConn1 -- Frame Sensor/RConn4
  PS-Simulink Converter5/LConn1 -- Frame Sensor/RConn7

== system nmm2d/Body Mechanics Layer/body sensor1 ==
  Frame Sensor : sm_lib/Frames and Transforms/Transform Sensor  MeasurementFrame=World  RotationSequence=XYX  SenseAngle=off  SenseAxis=off  SenseQ=off  SenseR=off  SenseRotationSequence=off  SenseOmegaX=off  SenseOmegaY=off  SenseOmegaZ=off  SenseOmega=off  SenseQDot=off  SenseRDot=off  SenseRotationSequenceDot=off  SenseAlphaX=off  SenseAlphaY=off  SenseAlphaZ=off  SenseAlpha=off  SenseQDDot=off  SenseRDDot=off  SenseX=on  SenseY=on  SenseZ=on  SenseXYZ=off  SenseRad=off  SenseAzim=off  SenseDist=off  SenseInc=off  SenseXDot=on  SenseYDot=on  SenseZDot=on  SenseXYZDot=off  SenseRadDot=off  SenseAzimDot=off  SenseDistDot=off  SenseIncDot=off  SenseXDDot=off  SenseYDDot=off  SenseZDDot=off  SenseXYZDDot=off  SenseRadDDot=off  SenseAzimDDot=off  SenseDistDDot=off  SenseIncDDot=off
  Mux : Mux  Inputs=3
  Mux1 : Mux  Inputs=3
  PS-Simulink Converter : nesl_utility/PS-Simulink Converter  PhysicalDomain=network_engine_domain  SubClassName=ps_output  LeftPortType=input  RightPortType=output  PseudoPeriodic=off  Frequencies=[]  VectorFormat=1-D array  Unit=m  AffineConversion=off
  PS-Simulink Converter1 : nesl_utility/PS-Simulink Converter  PhysicalDomain=network_engine_domain  SubClassName=ps_output  LeftPortType=input  RightPortType=output  PseudoPeriodic=off  Frequencies=[]  VectorFormat=1-D array  Unit=m  AffineConversion=off
  PS-Simulink Converter2 : nesl_utility/PS-Simulink Converter  PhysicalDomain=network_engine_domain  SubClassName=ps_output  LeftPortType=input  RightPortType=output  PseudoPeriodic=off  Frequencies=[]  VectorFormat=1-D array  Unit=m/s  AffineConversion=off
  PS-Simulink Converter3 : nesl_utility/PS-Simulink Converter  PhysicalDomain=network_engine_domain  SubClassName=ps_output  LeftPortType=input  RightPortType=output  PseudoPeriodic=off  Frequencies=[]  VectorFormat=1-D array  Unit=m/s  AffineConversion=off
  PS-Simulink Converter4 : nesl_utility/PS-Simulink Converter  PhysicalDomain=network_engine_domain  SubClassName=ps_output  LeftPortType=input  RightPortType=output  PseudoPeriodic=off  Frequencies=[]  VectorFormat=1-D array  Unit=m  AffineConversion=off
  PS-Simulink Converter5 : nesl_utility/PS-Simulink Converter  PhysicalDomain=network_engine_domain  SubClassName=ps_output  LeftPortType=input  RightPortType=output  PseudoPeriodic=off  Frequencies=[]  VectorFormat=1-D array  Unit=m/s  AffineConversion=off
  World Frame : sm_lib/Frames and Transforms/World Frame
  frame : PMIOPort  Side=Left
  p [m x3] : Outport
  v [m/s x3] : Outport  Port=2
  wires:
  PS-Simulink Converter5/1 -> Mux1/3
  PS-Simulink Converter4/1 -> Mux/3
  Mux/1 -> p [m x3]/1
  Mux1/1 -> v [m/s x3]/1
  PS-Simulink Converter3/1 -> Mux1/2
  PS-Simulink Converter2/1 -> Mux1/1
  PS-Simulink Converter/1 -> Mux/1
  PS-Simulink Converter1/1 -> Mux/2
  connections:
  PS-Simulink Converter5/LConn1 -- Frame Sensor/RConn7
  PS-Simulink Converter4/LConn1 -- Frame Sensor/RConn4
  PS-Simulink Converter3/LConn1 -- Frame Sensor/RConn6
  PS-Simulink Converter2/LConn1 -- Frame Sensor/RConn5
  PS-Simulink Converter1/LConn1 -- Frame Sensor/RConn3
  Frame Sensor/RConn2 -- PS-Simulink Converter/LConn1
  World Frame/RConn1 -- Frame Sensor/LConn1
  Frame Sensor/RConn1 -- frame/RConn1
